simulink model "CyberDog_Motor_FOC"  (R2025b)
settings: Solver=FixedStepDiscrete  StartTime=0.0  StopTime=inf  FixedStep=0.0001  RelTol=1e-3
InitFcn:
  | p = fileparts(get_param(bdroot,'FileName')); addpath(fullfile(p,'scripts')); motor_params;
undefined symbols (not defined in the file): Cogging_Lut_Angle, Cogging_Lut_V, CoggingFF_En, Curr_MaxOut, Curr_MinOut, CurrD_Ki, CurrD_Kp, CurrD_MaxOut, CurrD_MinOut, CurrQ_Ki, CurrQ_Kp, DeadComp_En, DeadComp_Lut_I, DeadComp_Lut_V, InvTwoPiPolePairs, InvVbus, MotorCfg, PLL_Ki, PLL_Kp, Pos_Kd, Pos_Kp, Pos_MaxOut, Pos_MinOut, Speed_Ki, Speed_Kp, Speed_MaxOut, Speed_MinOut, VmaxCoeff
libraries: slpidlib x4, mcbeeMathTransformLib x3, mcbcontrolslib x2, mcbsensorlessestimatorlib x1
settings Model: Creator=Baseline  LastModifiedBy=Baseline
settings DataIOCC: SaveOutput=off
settings OptimizationCC: DefaultParameterBehavior=Inlined  DefaultUnderspecifiedDataType=single  EnhancedBackFolding=on  PassReuseOutputArgsAs=Individual arguments  ZeroExternalMemoryAtStartup=off  ZeroInternalMemoryAtStartup=off  OptimizeBlockOrder=speed  DifferentSizesBufferReuse=on  OptimizationCustomize=off  EfficientTunableParamExpr=on
settings DebuggingCC: ParameterPrecisionLossMsg=none  ParameterTunabilityLossMsg=error
settings SFSimCC: MATLABDynamicMemAlloc=off
settings RTWCC: SystemTargetFile=ert.tlc  GenCodeOnly=on  GenerateMakefile=off  TemplateMakefile=ert_default_tmf  Description=Embedded Coder
settings CodeAppCC: ForceParamTrailComments=on  IgnoreCustomStorageClasses=off  OperatorAnnotations=on  SimulinkDataObjDesc=on  SFDataObjDesc=on  InsertBlockDesc=on
settings ERTTargetCC: ERTCustomFileTemplate=example_file_process.tlc  TargetLangStandard=C99 (ISO)  GenerateSampleERTMain=on

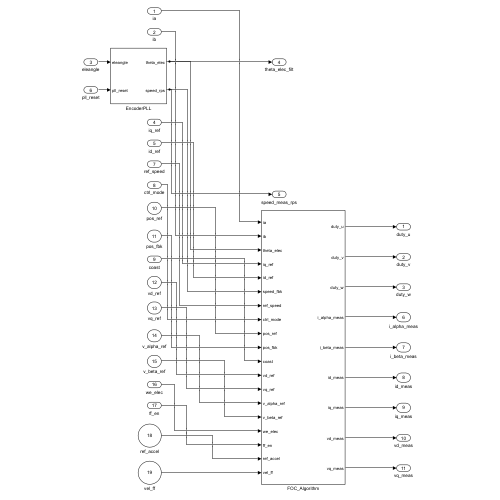
[thumbnail: Simulink's stored preview of the top-level diagram]
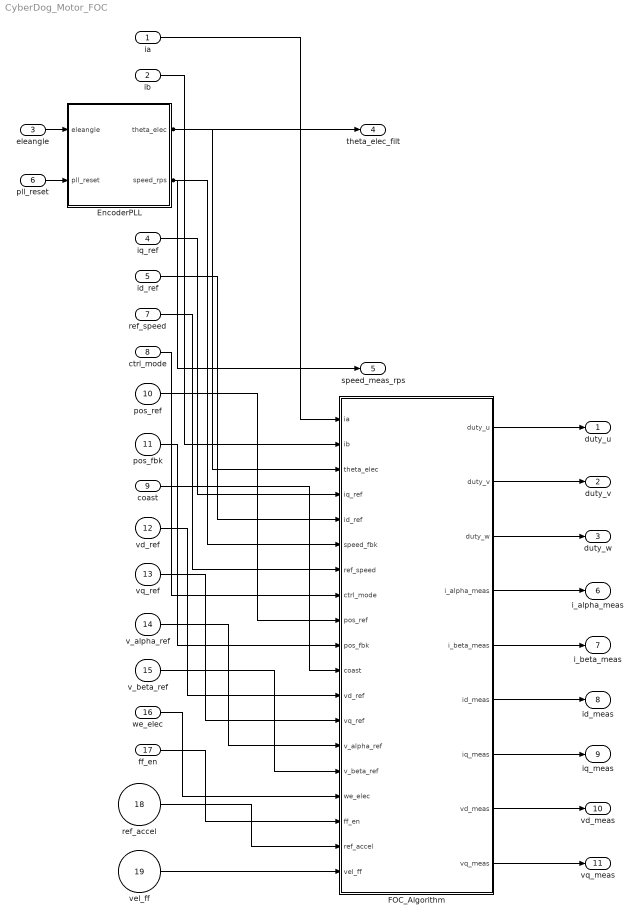
== system CyberDog_Motor_FOC ==
  ia : Inport  OutDataTypeStr=single  SampleTime=1e-4
  ib : Inport  Port=2  OutDataTypeStr=single  SampleTime=1e-4
  eleangle : Inport  Port=3  OutDataTypeStr=single  SampleTime=1e-4
  iq_ref : Inport  Port=4  OutDataTypeStr=single  SampleTime=1e-4
  id_ref : Inport  Port=5  OutDataTypeStr=single  SampleTime=1e-4
  pll_reset : Inport  Port=6  OutDataTypeStr=single  SampleTime=1e-4
  ref_speed : Inport  Port=7  OutDataTypeStr=single  SampleTime=1e-4
  ctrl_mode : Inport  Port=8  OutDataTypeStr=single  SampleTime=1e-4
  coast : Inport  Port=9  OutDataTypeStr=single
  pos_ref : Inport  Port=10  OutDataTypeStr=single
  pos_fbk : Inport  Port=11  OutDataTypeStr=single
  vd_ref : Inport  Port=12  OutDataTypeStr=single
  vq_ref : Inport  Port=13  OutDataTypeStr=single
  v_alpha_ref : Inport  Port=14  OutDataTypeStr=single
  v_beta_ref : Inport  Port=15  OutDataTypeStr=single
  we_elec : Inport  Port=16
  ff_en : Inport  Port=17
  ref_accel : Inport  Port=18
  vel_ff : Inport  Port=19
  EncoderPLL : Subsystem
  FOC_Algorithm : Subsystem
      settings: MinAlgLoopOccurrences=on
  duty_u : Outport  OutDataTypeStr=single
  duty_v : Outport  Port=2  OutDataTypeStr=single
  duty_w : Outport  Port=3  OutDataTypeStr=single
  theta_elec_filt : Outport  Port=4
  speed_meas_rps : Outport  Port=5
  i_alpha_meas : Outport  Port=6
  i_beta_meas : Outport  Port=7
  id_meas : Outport  Port=8
  iq_meas : Outport  Port=9
  vd_meas : Outport  Port=10
  vq_meas : Outport  Port=11
  wires:
  eleangle/1 -> EncoderPLL/1(eleangle)
  pll_reset/1 -> EncoderPLL/2(pll_reset)
  id_ref/1 -> FOC_Algorithm/5(id_ref)
  FOC_Algorithm/7(iq_meas) -> iq_meas/1
  EncoderPLL/1(theta_elec) -> theta_elec_filt/1, FOC_Algorithm/3(theta_elec)
  FOC_Algorithm/9(vq_meas) -> vq_meas/1
  FOC_Algorithm/5(i_beta_meas) -> i_beta_meas/1
  ia/1 -> FOC_Algorithm/1(ia)
  ib/1 -> FOC_Algorithm/2(ib)
  iq_ref/1 -> FOC_Algorithm/4(iq_ref)
  EncoderPLL/2(speed_rps) -> FOC_Algorithm/6(speed_fbk), speed_meas_rps/1
  coast/1 -> FOC_Algorithm/11(coast)
  ctrl_mode/1 -> FOC_Algorithm/8(ctrl_mode)
  ref_speed/1 -> FOC_Algorithm/7(ref_speed)
  pos_ref/1 -> FOC_Algorithm/9(pos_ref)
  FOC_Algorithm/8(vd_meas) -> vd_meas/1
  FOC_Algorithm/4(i_alpha_meas) -> i_alpha_meas/1
  pos_fbk/1 -> FOC_Algorithm/10(pos_fbk)
  vd_ref/1 -> FOC_Algorithm/12(vd_ref)
  FOC_Algorithm/1(duty_u) -> duty_u/1
  vq_ref/1 -> FOC_Algorithm/13(vq_ref)
  v_alpha_ref/1 -> FOC_Algorithm/14(v_alpha_ref)
  v_beta_ref/1 -> FOC_Algorithm/15(v_beta_ref)
  we_elec/1 -> FOC_Algorithm/16(we_elec)
  ff_en/1 -> FOC_Algorithm/17(ff_en)
  ref_accel/1 -> FOC_Algorithm/18(ref_accel)
  vel_ff/1 -> FOC_Algorithm/19(vel_ff)
  FOC_Algorithm/2(duty_v) -> duty_v/1
  FOC_Algorithm/3(duty_w) -> duty_w/1
  FOC_Algorithm/6(id_meas) -> id_meas/1

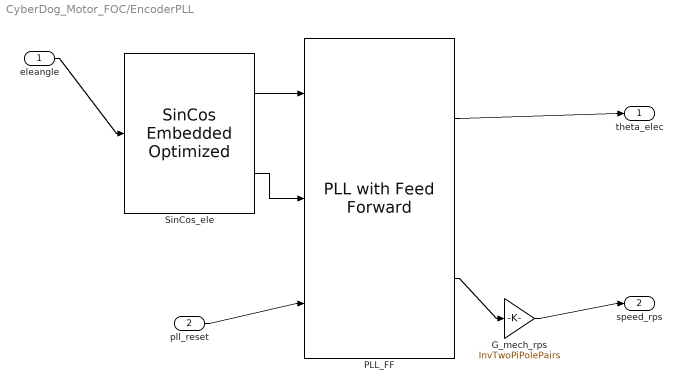
== system CyberDog_Motor_FOC/EncoderPLL ==
  eleangle : Inport
  pll_reset : Inport  Port=2
  G_mech_rps : Gain  Gain=InvTwoPiPolePairs
  PLL_FF : mcbsensorlessestimatorlib/PLL with Feed Forward  Normalization=off  ParameterBusInput=off  PosOut=Angular position  BlkSampleTime=1e-4  FreqRatio=1  MaximumApplicationFreq=7500  SpeedCutoffFreq=PLL_SpeedCutoffFreq  N_points=1024  Kp=PLL_Kp  Ki=PLL_Ki  PositionUnit=Radians  PositionDataType=single  FrequencyUnit=Radians/Sec  FrequencyDataType=single  TableDataType=single
      settings: LibrarySourceBlock=mcblib/Signal Management/PLL with Feed Forward
  SinCos_ele : mcbcontrolslib/SinCos Embedded Optimized  LabelModeActiveChoice=MCB_Sin  OptforProc=off  ApproximationMethod=None  UserApproxMethod=Lookup  ApproxStatus=None  InterpMethod=Linear point-slope  NumberOfDataPoints=16  NumberOfIterations=11  RemoveProtectionAgainstOutOfRangeInput=off  TableDataTypeStr=Inherit: Inherit via input  AngleInput=Radians  ThetaDataType=single  N_points=1024  DatatypeInput=Inherit from input  Datatype=single
  theta_elec : Outport
  speed_rps : Outport  Port=2
  wires:
  pll_reset/1 -> PLL_FF/3
  PLL_FF/1 -> theta_elec/1
  PLL_FF/2 -> G_mech_rps/1
  G_mech_rps/1 -> speed_rps/1
  eleangle/1 -> SinCos_ele/1
  SinCos_ele/1 -> PLL_FF/1
  SinCos_ele/2 -> PLL_FF/2

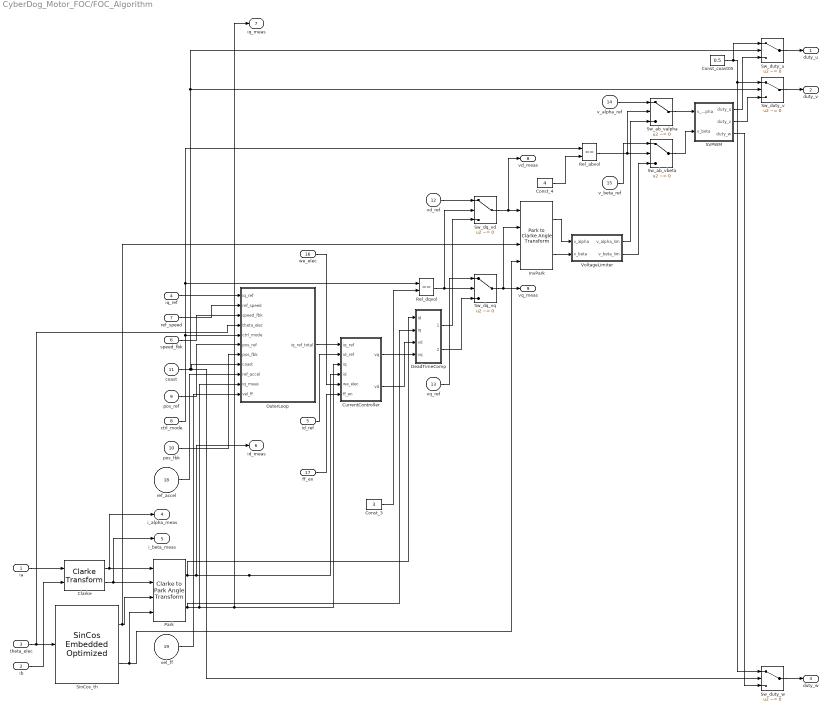
== system CyberDog_Motor_FOC/FOC_Algorithm ==
  ia : Inport
  ib : Inport  Port=2
  theta_elec : Inport  Port=3  OutDataTypeStr=single
  iq_ref : Inport  Port=4  OutDataTypeStr=single
  id_ref : Inport  Port=5  OutDataTypeStr=single
  speed_fbk : Inport  Port=6  OutDataTypeStr=single
  ref_speed : Inport  Port=7  OutDataTypeStr=single
  ctrl_mode : Inport  Port=8  OutDataTypeStr=single
  pos_ref : Inport  Port=9  OutDataTypeStr=single
  pos_fbk : Inport  Port=10  OutDataTypeStr=single
  coast : Inport  Port=11  OutDataTypeStr=single
  vd_ref : Inport  Port=12  OutDataTypeStr=single
  vq_ref : Inport  Port=13  OutDataTypeStr=single
  v_alpha_ref : Inport  Port=14  OutDataTypeStr=single
  v_beta_ref : Inport  Port=15  OutDataTypeStr=single
  we_elec : Inport  Port=16
  ff_en : Inport  Port=17
  ref_accel : Inport  Port=18
  vel_ff : Inport  Port=19
  Clarke : mcbeeMathTransformLib/Clarke Transform  VariantControl=Variant2  PowerInvariant=off  UseWithEmbedded=on  PhaseInput=Two inputs
      settings: LibrarySourceBlock=mcbfoclib/Field-Oriented Current Controller/Clarke Transform
  Const_3 : Constant  Value=3  OutDataTypeStr=single
  Const_4 : Constant  Value=4  OutDataTypeStr=single
  Const_coast05 : Constant  Value=0.5  OutDataTypeStr=single
  CurrentController : Subsystem
  DeadTimeComp : Subsystem
  InvPark : mcbeeMathTransformLib/Park to Clarke Angle Transform  AxisAlignment=D-axis  UseWithEmbedded=on  PhaseInput=Two inputs  ThetaInput=Sine and Cosine electrical position  AngleInput=Per-unit  N_points=1024
      settings: LibrarySourceBlock=mcbfoclib/Field-Oriented Current Controller/Inverse Park Transform
  OuterLoop : Subsystem
  Park : mcbeeMathTransformLib/Clarke to Park Angle Transform  AxisAlignment=D-axis  UseWithEmbedded=on  PhaseInput=Two inputs  ThetaInput=Sine and Cosine electrical position  AngleInput=Radians  N_points=1024
      settings: LibrarySourceBlock=mcbfoclib/Field-Oriented Current Controller/Park Transform
  Rel_abvol : RelationalOperator  Operator===  OutDataTypeStr=boolean  RndMeth=Simplest  InputSameDT=off
  Rel_dqvol : RelationalOperator  Operator===  OutDataTypeStr=boolean  RndMeth=Simplest  InputSameDT=off
  SVPWM : Subsystem
  SinCos_th : mcbcontrolslib/SinCos Embedded Optimized  LabelModeActiveChoice=MCB_Sin  OptforProc=off  ApproximationMethod=None  UserApproxMethod=Lookup  ApproxStatus=None  InterpMethod=Linear point-slope  NumberOfDataPoints=16  NumberOfIterations=11  RemoveProtectionAgainstOutOfRangeInput=off  TableDataTypeStr=Inherit: Inherit via input  AngleInput=Radians  ThetaDataType=single  N_points=1024  DatatypeInput=Inherit from input  Datatype=single
  Sw_ab_valpha : Switch  Criteria=u2 ~= 0  SaturateOnIntegerOverflow=off  InputSameDT=off
  Sw_ab_vbeta : Switch  Criteria=u2 ~= 0  SaturateOnIntegerOverflow=off  InputSameDT=off
  Sw_dq_vd : Switch  Criteria=u2 ~= 0  SaturateOnIntegerOverflow=off  InputSameDT=off
  Sw_dq_vq : Switch  Criteria=u2 ~= 0  SaturateOnIntegerOverflow=off  InputSameDT=off
  Sw_duty_u : Switch  Criteria=u2 ~= 0  SaturateOnIntegerOverflow=off  InputSameDT=off
  Sw_duty_v : Switch  Criteria=u2 ~= 0  SaturateOnIntegerOverflow=off  InputSameDT=off
  Sw_duty_w : Switch  Criteria=u2 ~= 0  SaturateOnIntegerOverflow=off  InputSameDT=off
  VoltageLimiter : Subsystem
  duty_u : Outport
  duty_v : Outport  Port=2
  duty_w : Outport  Port=3
  i_alpha_meas : Outport  Port=4
  i_beta_meas : Outport  Port=5
  id_meas : Outport  Port=6
  iq_meas : Outport  Port=7
  vd_meas : Outport  Port=8
  vq_meas : Outport  Port=9
  wires:
  ib/1 -> Clarke/2
  VoltageLimiter/2(v_beta_lim) -> Sw_ab_vbeta/3
  ctrl_mode/1 -> Rel_dqvol/1, Rel_abvol/1, OuterLoop/5(ctrl_mode)
  ia/1 -> Clarke/1
  Clarke/1 -> Park/1, i_alpha_meas/1
  vq_ref/1 -> Sw_dq_vq/1
  theta_elec/1 -> OuterLoop/4(theta_elec), SinCos_th/1
  iq_ref/1 -> OuterLoop/1(iq_ref)
  id_ref/1 -> CurrentController/2(id_ref)
  SinCos_th/1 -> InvPark/3, Park/3
  InvPark/1 -> VoltageLimiter/1(v_alpha)
  Clarke/2 -> Park/2, i_beta_meas/1
  Sw_dq_vq/1 -> vq_meas/1, InvPark/2
  SinCos_th/2 -> InvPark/4, Park/4
  ref_speed/1 -> OuterLoop/2(ref_speed)
  DeadTimeComp/1(vd_out) -> Sw_dq_vd/3
  speed_fbk/1 -> OuterLoop/3(speed_fbk)
  coast/1 -> Sw_duty_w/2, OuterLoop/8(coast), Sw_duty_u/2, Sw_duty_v/2
  pos_ref/1 -> OuterLoop/6(pos_ref)
  pos_fbk/1 -> OuterLoop/7(pos_fbk)
  ref_accel/1 -> OuterLoop/9(ref_accel)
  Park/1 -> CurrentController/4(id), id_meas/1, DeadTimeComp/1(id)
  Park/2 -> iq_meas/1, CurrentController/3(iq), OuterLoop/10(iq_meas), DeadTimeComp/2(iq)
  vel_ff/1 -> OuterLoop/11(vel_ff)
  SVPWM/1(duty_u) -> Sw_duty_u/3
  we_elec/1 -> CurrentController/5(we_elec)
  Sw_duty_u/1 -> duty_u/1
  Const_coast05/1 -> Sw_duty_v/1, Sw_duty_w/1, Sw_duty_u/1
  Const_3/1 -> Rel_dqvol/2
  OuterLoop/1(iq_ref_total) -> CurrentController/1(iq_ref)
  ff_en/1 -> CurrentController/6(ff_en)
  CurrentController/1(vq) -> DeadTimeComp/4(vq)
  v_beta_ref/1 -> Sw_ab_vbeta/1
  DeadTimeComp/2(vq_out) -> Sw_dq_vq/3
  CurrentController/2(vd) -> DeadTimeComp/3(vd)
  vd_ref/1 -> Sw_dq_vd/1
  Rel_dqvol/1 -> Sw_dq_vd/2, Sw_dq_vq/2
  Sw_dq_vd/1 -> vd_meas/1, InvPark/1
  Const_4/1 -> Rel_abvol/2
  InvPark/2 -> VoltageLimiter/2(v_beta)
  v_alpha_ref/1 -> Sw_ab_valpha/1
  Sw_duty_v/1 -> duty_v/1
  Rel_abvol/1 -> Sw_ab_vbeta/2, Sw_ab_valpha/2
  VoltageLimiter/1(v_alpha_lim) -> Sw_ab_valpha/3
  Sw_ab_valpha/1 -> SVPWM/1(v_alpha)
  Sw_ab_vbeta/1 -> SVPWM/2(v_beta)
  SVPWM/2(duty_v) -> Sw_duty_v/3
  SVPWM/3(duty_w) -> Sw_duty_w/3
  Sw_duty_w/1 -> duty_w/1

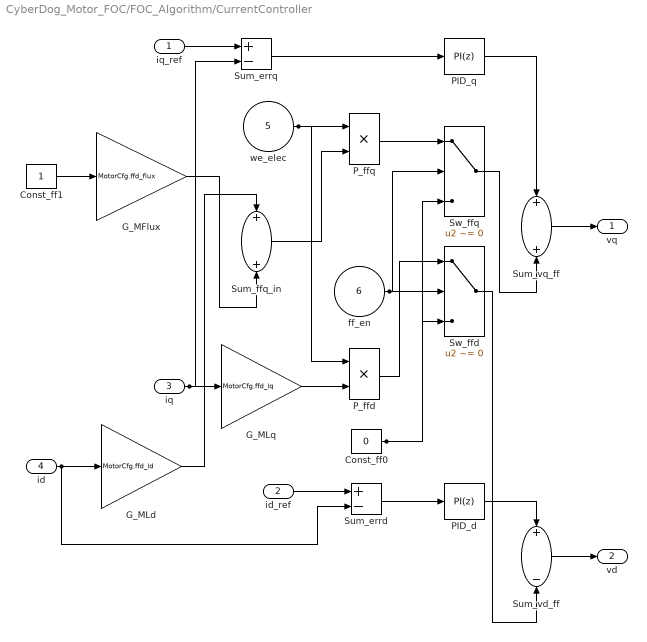
== system CyberDog_Motor_FOC/FOC_Algorithm/CurrentController ==
  iq_ref : Inport  OutDataTypeStr=single
  id_ref : Inport  Port=2  OutDataTypeStr=single
  iq : Inport  Port=3
  id : Inport  Port=4
  we_elec : Inport  Port=5
  ff_en : Inport  Port=6
  Const_ff0 : Constant  Value=0  OutDataTypeStr=single
  Const_ff1 : Constant  OutDataTypeStr=single
  G_MFlux : Gain  Gain=MotorCfg.ffd_flux  OutDataTypeStr=single
  G_MLd : Gain  Gain=MotorCfg.ffd_ld  OutDataTypeStr=single
  G_MLq : Gain  Gain=MotorCfg.ffd_lq  OutDataTypeStr=single
  PID_d : slpidlib/PID Controller  Controller=PI  Form=Parallel  TimeDomain=Discrete-time  UseExternalTs=off  SampleTime=1e-4  IntegratorMethod=Forward Euler  FilterMethod=Forward Euler  ControllerParametersSource=internal  P=CurrD_Kp  I=CurrD_Ki  UseKiTs=on  D=0  UseExternalDerivativeSource=off  N=100  UseFilter=on  TunerSelectOption=Transfer Function Based (PID Tuner App)  InitialConditionSource=internal  InitialConditionForIntegrator=0  InitialConditionForFilter=0  DifferentiatorICPrevScaledInput=0  ExternalReset=none  TrackingMode=off  Kt=1  LimitOutput=on  SatLimitsSource=internal  UpperSaturationLimit=CurrD_MaxOut  LowerSaturationLimit=CurrD_MinOut  LinearizeAsGain=on  AntiWindupMode=back-calculation  Kb=1  LimitIntegrator=on  UpperIntegratorSaturationLimit=CurrD_MaxOut  LowerIntegratorSaturationLimit=CurrD_MinOut  POutMin=[]  POutMax=[]  IOutMin=[]  IOutMax=[]  DOutMin=[]  DOutMax=[]  NOutMin=[]  NOutMax=[]  SumOutMin=[]  SumOutMax=[]  SaturationOutMin=[]  SaturationOutMax=[]  PParamDataTypeStr=single  PParamMin=[]  PParamMax=[]  IParamDataTypeStr=single  IParamMin=[]  IParamMax=[]  DParamMin=[]  DParamMax=[]  NParamMin=[]  NParamMax=[]  KbParamDataTypeStr=single  KbParamMin=[]  KbParamMax=[]  KtParamMin=[]  KtParamMax=[]  KbOutDataTypeStr=single  KbOutMin=[]  KbOutMax=[]  KtOutMin=[]  KtOutMax=[]  IntegratorOutMin=[]  IntegratorOutMax=[]  FilterOutMin=[]  FilterOutMax=[]  SumI1OutMin=[]  SumI1OutMax=[]  SumI2OutDataTypeStr=single  SumI2OutMin=[]  SumI2OutMax=[]  SumI3OutMin=[]  SumI3OutMax=[]  SumI4OutMin=[]  SumI4OutMax=[]  SumDOutMin=[]  SumDOutMax=[]  DifferentiatorOutMin=[]  DifferentiatorOutMax=[]  FilterDiffOutCoefMin=[]  FilterDiffOutCoefMax=[]  ReciprocalOutMin=[]  ReciprocalOutMax=[]  SumDenOutMin=[]  SumDenOutMax=[]  SumNumOutMin=[]  SumNumOutMax=[]  DivideOutMin=[]  DivideOutMax=[]  UdiffTsProdOutMin=[]  UdiffTsProdOutMax=[]  NTsProdOutMin=[]  NTsProdOutMax=[]  UintegralTsProdOutMin=[]  UintegralTsProdOutMax=[]  UngainTsProdOutMin=[]  UngainTsProdOutMax=[]  ClampingZeroOutDataTypeStr=Inherit: Inherit via back propagation  ClampingZeroOutMin=[]  ClampingZeroOutMax=[]  FilterDenConstantOutDataTypeStr=Inherit: Inherit via back propagation  FilterDenConstantOutMin=[]  FilterDenConstantOutMax=[]  PCopyOutDataTypeStr=Inherit: Inherit via back propagation  PCopyOutMin=[]  PCopyOutMax=[]  NCopyOutDataTypeStr=Inherit: Inherit via back propagation  NCopyOutMin=[]  NCopyOutMax=[]  IntegratorContinuousStateAttributes=''  IntegratorStateMustResolveToSignalObject=off  IntegratorRTWStateStorageClass=Auto  FilterContinuousStateAttributes=''  FilterStateMustResolveToSignalObject=off  FilterRTWStateStorageClass=Auto  ParallelPVariant=InternalParameters  IdealPVariant=Disabled  IVariant=InternalParameters  DVariant=Disabled  IntegratorVariant=Discrete  SatVariant=Enabled  AWVariant=BackCalculation  PCopyVariant=Disabled  TRVariant=Disabled  FdbkBlocksVariant=Forward  IdealPFdbkVariant=Disabled  SatFdbkVariant=Disabled  DerivativeFilterVariant=Disabled  NVariant=Disabled  NCopyVariant=Disabled_SignalSpec  FilterICVariant=Disabled  IntegratorICVariant=InternalICs  ExternalResetVariant=Disabled  TRSumVariant=Passthrough  SumFdbkVariant=Disabled  SumVariant=Sum_PI  TsampFilterVariant=InternalTs  TsampNgainVariant=Passthrough  TsampIntegralVariant=Disabled_SignalSpec  ExternalSaturationOutDataTypeStr=Inherit: Same as second input  DerivativeSourceVariant=Disabled  PreIntVariant=InternalPreInt
  PID_q : slpidlib/PID Controller  Controller=PI  Form=Parallel  TimeDomain=Discrete-time  UseExternalTs=off  SampleTime=1e-4  IntegratorMethod=Forward Euler  FilterMethod=Forward Euler  ControllerParametersSource=internal  P=CurrQ_Kp  I=CurrQ_Ki  UseKiTs=on  D=0  UseExternalDerivativeSource=off  N=100  UseFilter=on  TunerSelectOption=Transfer Function Based (PID Tuner App)  InitialConditionSource=internal  InitialConditionForIntegrator=0  InitialConditionForFilter=0  DifferentiatorICPrevScaledInput=0  ExternalReset=none  TrackingMode=off  Kt=1  LimitOutput=on  SatLimitsSource=internal  UpperSaturationLimit=Curr_MaxOut  LowerSaturationLimit=Curr_MinOut  LinearizeAsGain=on  AntiWindupMode=back-calculation  Kb=1  LimitIntegrator=on  UpperIntegratorSaturationLimit=Curr_MaxOut  LowerIntegratorSaturationLimit=Curr_MinOut  POutMin=[]  POutMax=[]  IOutMin=[]  IOutMax=[]  DOutMin=[]  DOutMax=[]  NOutMin=[]  NOutMax=[]  SumOutMin=[]  SumOutMax=[]  SaturationOutMin=[]  SaturationOutMax=[]  PParamDataTypeStr=single  PParamMin=[]  PParamMax=[]  IParamDataTypeStr=single  IParamMin=[]  IParamMax=[]  DParamMin=[]  DParamMax=[]  NParamMin=[]  NParamMax=[]  KbParamDataTypeStr=single  KbParamMin=[]  KbParamMax=[]  KtParamMin=[]  KtParamMax=[]  KbOutDataTypeStr=single  KbOutMin=[]  KbOutMax=[]  KtOutMin=[]  KtOutMax=[]  IntegratorOutMin=[]  IntegratorOutMax=[]  FilterOutMin=[]  FilterOutMax=[]  SumI1OutMin=[]  SumI1OutMax=[]  SumI2OutDataTypeStr=single  SumI2OutMin=[]  SumI2OutMax=[]  SumI3OutMin=[]  SumI3OutMax=[]  SumI4OutMin=[]  SumI4OutMax=[]  SumDOutMin=[]  SumDOutMax=[]  DifferentiatorOutMin=[]  DifferentiatorOutMax=[]  FilterDiffOutCoefMin=[]  FilterDiffOutCoefMax=[]  ReciprocalOutMin=[]  ReciprocalOutMax=[]  SumDenOutMin=[]  SumDenOutMax=[]  SumNumOutMin=[]  SumNumOutMax=[]  DivideOutMin=[]  DivideOutMax=[]  UdiffTsProdOutMin=[]  UdiffTsProdOutMax=[]  NTsProdOutMin=[]  NTsProdOutMax=[]  UintegralTsProdOutMin=[]  UintegralTsProdOutMax=[]  UngainTsProdOutMin=[]  UngainTsProdOutMax=[]  ClampingZeroOutDataTypeStr=Inherit: Inherit via back propagation  ClampingZeroOutMin=[]  ClampingZeroOutMax=[]  FilterDenConstantOutDataTypeStr=Inherit: Inherit via back propagation  FilterDenConstantOutMin=[]  FilterDenConstantOutMax=[]  PCopyOutDataTypeStr=Inherit: Inherit via back propagation  PCopyOutMin=[]  PCopyOutMax=[]  NCopyOutDataTypeStr=Inherit: Inherit via back propagation  NCopyOutMin=[]  NCopyOutMax=[]  IntegratorContinuousStateAttributes=''  IntegratorStateMustResolveToSignalObject=off  IntegratorRTWStateStorageClass=Auto  FilterContinuousStateAttributes=''  FilterStateMustResolveToSignalObject=off  FilterRTWStateStorageClass=Auto  ParallelPVariant=InternalParameters  IdealPVariant=Disabled  IVariant=InternalParameters  DVariant=Disabled  IntegratorVariant=Discrete  SatVariant=Enabled  AWVariant=BackCalculation  PCopyVariant=Disabled  TRVariant=Disabled  FdbkBlocksVariant=Forward  IdealPFdbkVariant=Disabled  SatFdbkVariant=Disabled  DerivativeFilterVariant=Disabled  NVariant=Disabled  NCopyVariant=Disabled_SignalSpec  FilterICVariant=Disabled  IntegratorICVariant=InternalICs  ExternalResetVariant=Disabled  TRSumVariant=Passthrough  SumFdbkVariant=Disabled  SumVariant=Sum_PI  TsampFilterVariant=InternalTs  TsampNgainVariant=Passthrough  TsampIntegralVariant=Disabled_SignalSpec  ExternalSaturationOutDataTypeStr=Inherit: Same as second input  DerivativeSourceVariant=Disabled  PreIntVariant=InternalPreInt
  P_ffd : Product  OutDataTypeStr=single
  P_ffq : Product  OutDataTypeStr=single
  Sum_errd : Sum  Inputs=+-
  Sum_errq : Sum  Inputs=+-
  Sum_ffq_in : Sum  OutDataTypeStr=single
  Sum_vd_ff : Sum  Inputs=+-  OutDataTypeStr=single
  Sum_vq_ff : Sum  OutDataTypeStr=single
  Sw_ffd : Switch  Criteria=u2 ~= 0  OutDataTypeStr=single
  Sw_ffq : Switch  Criteria=u2 ~= 0  OutDataTypeStr=single
  vq : Outport
  vd : Outport  Port=2
  wires:
  Sum_errq/1 -> PID_q/1
  G_MLd/1 -> Sum_ffq_in/1
  Const_ff1/1 -> G_MFlux/1
  G_MFlux/1 -> Sum_ffq_in/2
  id/1 -> Sum_errd/2, G_MLd/1
  iq_ref/1 -> Sum_errq/1
  iq/1 -> G_MLq/1, Sum_errq/2
  we_elec/1 -> P_ffd/1, P_ffq/1
  Const_ff0/1 -> Sw_ffd/3, Sw_ffq/3
  Sum_ffq_in/1 -> P_ffq/2
  G_MLq/1 -> P_ffd/2
  id_ref/1 -> Sum_errd/1
  P_ffd/1 -> Sw_ffd/1
  P_ffq/1 -> Sw_ffq/1
  ff_en/1 -> Sw_ffd/2, Sw_ffq/2
  Sum_errd/1 -> PID_d/1
  PID_q/1 -> Sum_vq_ff/1
  Sw_ffq/1 -> Sum_vq_ff/2
  Sw_ffd/1 -> Sum_vd_ff/2
  PID_d/1 -> Sum_vd_ff/1
  Sum_vd_ff/1 -> vd/1
  Sum_vq_ff/1 -> vq/1

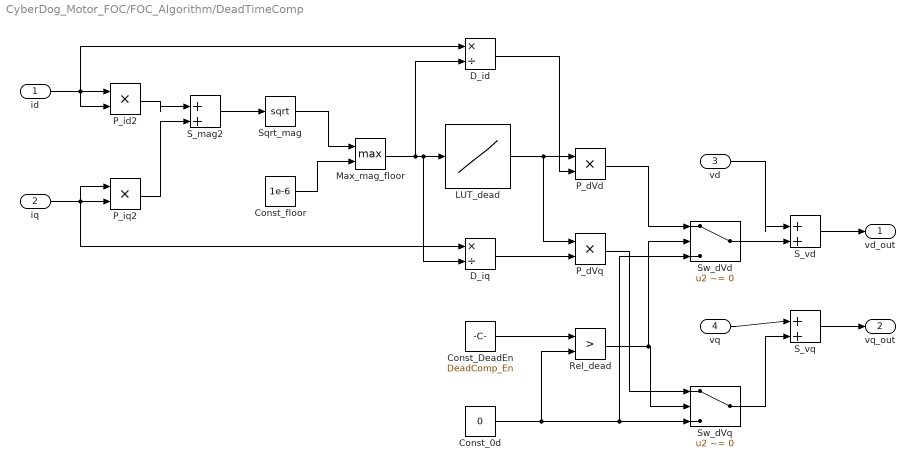
== system CyberDog_Motor_FOC/FOC_Algorithm/DeadTimeComp ==
  id : Inport
  iq : Inport  Port=2
  vd : Inport  Port=3
  vq : Inport  Port=4
  Const_0d : Constant  Value=0  OutDataTypeStr=single
  Const_DeadEn : Constant  Value=DeadComp_En  OutDataTypeStr=single
  Const_floor : Constant  Value=1e-6  OutDataTypeStr=single
  D_id : Product  Inputs=*/  OutDataTypeStr=single
  D_iq : Product  Inputs=*/  OutDataTypeStr=single
  LUT_dead : Lookup_n-D  NumberOfTableDimensions=1  BreakpointsForDimension1=DeadComp_Lut_I  Table=DeadComp_Lut_V  InternalRulePriority=Speed  OutDataTypeStr=single  RndMeth=Simplest
  Max_mag_floor : MinMax  Function=max  Inputs=2  OutDataTypeStr=single
  P_dVd : Product  Inputs=**  OutDataTypeStr=single
  P_dVq : Product  Inputs=**  OutDataTypeStr=single
  P_id2 : Product  Inputs=**  OutDataTypeStr=single
  P_iq2 : Product  Inputs=**  OutDataTypeStr=single
  Rel_dead : RelationalOperator  Operator=>  OutDataTypeStr=boolean  RndMeth=Simplest  InputSameDT=off
  S_mag2 : Sum  Inputs=|++  OutDataTypeStr=single
  S_vd : Sum  Inputs=|++
  S_vq : Sum  Inputs=|++
  Sqrt_mag : Sqrt  OutDataTypeStr=single
  Sw_dVd : Switch  Criteria=u2 ~= 0  OutDataTypeStr=single  SaturateOnIntegerOverflow=off  InputSameDT=off
  Sw_dVq : Switch  Criteria=u2 ~= 0  OutDataTypeStr=single  SaturateOnIntegerOverflow=off  InputSameDT=off
  vd_out : Outport
  vq_out : Outport  Port=2
  wires:
  S_vq/1 -> vq_out/1
  S_vd/1 -> vd_out/1
  Sw_dVq/1 -> S_vq/2
  vq/1 -> S_vq/1
  Sw_dVd/1 -> S_vd/2
  vd/1 -> S_vd/1
  Const_DeadEn/1 -> Rel_dead/1
  P_dVq/1 -> Sw_dVq/1
  Const_0d/1 -> Sw_dVd/3, Sw_dVq/3, Rel_dead/2
  Rel_dead/1 -> Sw_dVd/2, Sw_dVq/2
  P_dVd/1 -> Sw_dVd/1
  D_iq/1 -> P_dVq/2
  D_id/1 -> P_dVd/2
  LUT_dead/1 -> P_dVd/1, P_dVq/1
  Max_mag_floor/1 -> LUT_dead/1, D_iq/2, D_id/2
  Const_floor/1 -> Max_mag_floor/2
  Sqrt_mag/1 -> Max_mag_floor/1
  S_mag2/1 -> Sqrt_mag/1
  P_iq2/1 -> S_mag2/2
  P_id2/1 -> S_mag2/1
  iq/1 -> D_iq/1, P_iq2/1, P_iq2/2
  id/1 -> P_id2/1, P_id2/2, D_id/1

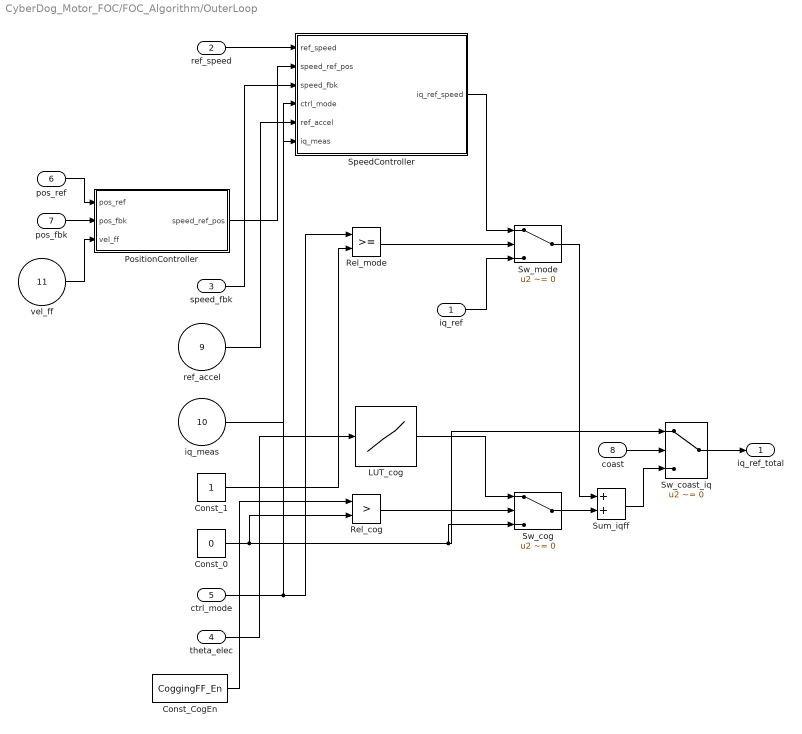
== system CyberDog_Motor_FOC/FOC_Algorithm/OuterLoop ==
  iq_ref : Inport  OutDataTypeStr=single
  ref_speed : Inport  Port=2  OutDataTypeStr=single
  speed_fbk : Inport  Port=3  OutDataTypeStr=single
  theta_elec : Inport  Port=4  OutDataTypeStr=single
  ctrl_mode : Inport  Port=5  OutDataTypeStr=single
  pos_ref : Inport  Port=6  OutDataTypeStr=single
  pos_fbk : Inport  Port=7  OutDataTypeStr=single
  coast : Inport  Port=8  OutDataTypeStr=single
  ref_accel : Inport  Port=9
  iq_meas : Inport  Port=10
  vel_ff : Inport  Port=11
  Const_0 : Constant  Value=0  OutDataTypeStr=single
  Const_1 : Constant  OutDataTypeStr=single
  Const_CogEn : Constant  Value=CoggingFF_En  OutDataTypeStr=single
  LUT_cog : Lookup_n-D  NumberOfTableDimensions=1  BreakpointsForDimension1=Cogging_Lut_Angle  Table=Cogging_Lut_V  InternalRulePriority=Speed  OutDataTypeStr=single  RndMeth=Simplest
  PositionController : Subsystem
  Rel_cog : RelationalOperator  Operator=>  OutDataTypeStr=boolean  RndMeth=Simplest  InputSameDT=off
  Rel_mode : RelationalOperator  OutDataTypeStr=boolean  RndMeth=Simplest  InputSameDT=off
  SpeedController : Subsystem
  Sum_iqff : Sum  OutDataTypeStr=single
  Sw_coast_iq : Switch  Criteria=u2 ~= 0  SaturateOnIntegerOverflow=off  InputSameDT=off
  Sw_cog : Switch  Criteria=u2 ~= 0  OutDataTypeStr=single  SaturateOnIntegerOverflow=off  InputSameDT=off
  Sw_mode : Switch  Criteria=u2 ~= 0  OutDataTypeStr=single  SaturateOnIntegerOverflow=off  InputSameDT=off
  iq_ref_total : Outport
  wires:
  Sw_cog/1 -> Sum_iqff/2
  pos_fbk/1 -> PositionController/2(pos_fbk)
  speed_fbk/1 -> SpeedController/3(speed_fbk)
  pos_ref/1 -> PositionController/1(pos_ref)
  ref_speed/1 -> SpeedController/1(ref_speed)
  vel_ff/1 -> PositionController/3(vel_ff)
  LUT_cog/1 -> Sw_cog/1
  iq_meas/1 -> SpeedController/6(iq_meas)
  PositionController/1(speed_ref_pos) -> SpeedController/2(speed_ref_pos)
  ref_accel/1 -> SpeedController/5(ref_accel)
  Const_1/1 -> Rel_mode/2
  Sw_mode/1 -> Sum_iqff/1
  Const_0/1 -> Sw_cog/3, Sw_coast_iq/1, Rel_cog/2
  iq_ref/1 -> Sw_mode/3
  ctrl_mode/1 -> Rel_mode/1, SpeedController/4(ctrl_mode)
  theta_elec/1 -> LUT_cog/1
  Const_CogEn/1 -> Rel_cog/1
  SpeedController/1(iq_ref_speed) -> Sw_mode/1
  Rel_mode/1 -> Sw_mode/2
  Rel_cog/1 -> Sw_cog/2
  coast/1 -> Sw_coast_iq/2
  Sum_iqff/1 -> Sw_coast_iq/3
  Sw_coast_iq/1 -> iq_ref_total/1

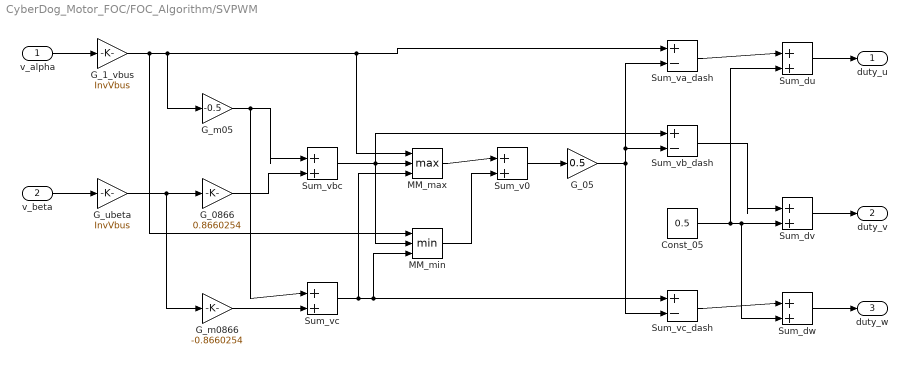
== system CyberDog_Motor_FOC/FOC_Algorithm/SVPWM ==
  v_alpha : Inport  OutDataTypeStr=single
  v_beta : Inport  Port=2  OutDataTypeStr=single
  Const_05 : Constant  Value=0.5  OutDataTypeStr=single
  G_05 : Gain  Gain=0.5  ParamDataTypeStr=single  OutDataTypeStr=single
  G_0866 : Gain  Gain=0.8660254  ParamDataTypeStr=single  OutDataTypeStr=single
  G_1_vbus : Gain  Gain=InvVbus  ParamDataTypeStr=single  OutDataTypeStr=single
  G_m05 : Gain  Gain=-0.5  ParamDataTypeStr=single  OutDataTypeStr=single
  G_m0866 : Gain  Gain=-0.8660254  ParamDataTypeStr=single  OutDataTypeStr=single
  G_ubeta : Gain  Gain=InvVbus  ParamDataTypeStr=single  OutDataTypeStr=single
  MM_max : MinMax  Function=max  Inputs=3  OutDataTypeStr=single
  MM_min : MinMax  Inputs=3  OutDataTypeStr=single
  Sum_du : Sum  Inputs=|++  OutDataTypeStr=single
  Sum_dv : Sum  Inputs=|++  OutDataTypeStr=single
  Sum_dw : Sum  Inputs=|++  OutDataTypeStr=single
  Sum_v0 : Sum  Inputs=|++  OutDataTypeStr=single
  Sum_va_dash : Sum  Inputs=+-  OutDataTypeStr=single
  Sum_vb_dash : Sum  Inputs=+-  OutDataTypeStr=single
  Sum_vbc : Sum  Inputs=|++  OutDataTypeStr=single
  Sum_vc : Sum  Inputs=|++  OutDataTypeStr=single
  Sum_vc_dash : Sum  Inputs=+-  OutDataTypeStr=single
  duty_u : Outport
  duty_v : Outport  Port=2
  duty_w : Outport  Port=3
  wires:
  Sum_dw/1 -> duty_w/1
  Sum_dv/1 -> duty_v/1
  Sum_du/1 -> duty_u/1
  Sum_vc_dash/1 -> Sum_dw/1
  Sum_vb_dash/1 -> Sum_dv/1
  Const_05/1 -> Sum_dv/2, Sum_dw/2, Sum_du/2
  Sum_va_dash/1 -> Sum_du/1
  G_05/1 -> Sum_va_dash/2, Sum_vb_dash/2, Sum_vc_dash/2
  Sum_v0/1 -> G_05/1
  MM_min/1 -> Sum_v0/2
  MM_max/1 -> Sum_v0/1
  Sum_vc/1 -> Sum_vc_dash/1, MM_min/3, MM_max/3
  Sum_vbc/1 -> MM_max/2, MM_min/2, Sum_vb_dash/1
  G_m0866/1 -> Sum_vc/2
  G_0866/1 -> Sum_vbc/2
  G_m05/1 -> Sum_vbc/1, Sum_vc/1
  G_ubeta/1 -> G_0866/1, G_m0866/1
  G_1_vbus/1 -> Sum_va_dash/1, MM_max/1, G_m05/1, MM_min/1
  v_beta/1 -> G_ubeta/1
  v_alpha/1 -> G_1_vbus/1

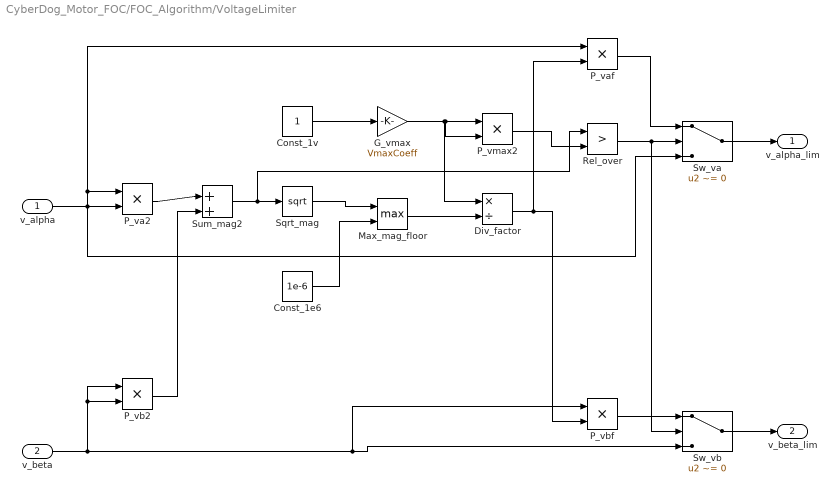
== system CyberDog_Motor_FOC/FOC_Algorithm/VoltageLimiter ==
  v_alpha : Inport
  v_beta : Inport  Port=2
  Const_1e6 : Constant  Value=1e-6  OutDataTypeStr=single
  Const_1v : Constant  OutDataTypeStr=single
  Div_factor : Product  Inputs=*/  OutDataTypeStr=single
  G_vmax : Gain  Gain=VmaxCoeff  ParamDataTypeStr=single  OutDataTypeStr=single
  Max_mag_floor : MinMax  Function=max  Inputs=2  OutDataTypeStr=single
  P_va2 : Product  Inputs=**  OutDataTypeStr=single
  P_vaf : Product  Inputs=**  OutDataTypeStr=single
  P_vb2 : Product  Inputs=**  OutDataTypeStr=single
  P_vbf : Product  Inputs=**  OutDataTypeStr=single
  P_vmax2 : Product  Inputs=**  OutDataTypeStr=single
  Rel_over : RelationalOperator  Operator=>  OutDataTypeStr=boolean  RndMeth=Simplest  InputSameDT=off
  Sqrt_mag : Sqrt  OutDataTypeStr=single
  Sum_mag2 : Sum  Inputs=|++  OutDataTypeStr=single
  Sw_va : Switch  Criteria=u2 ~= 0  OutDataTypeStr=single  SaturateOnIntegerOverflow=off  InputSameDT=off
  Sw_vb : Switch  Criteria=u2 ~= 0  OutDataTypeStr=single  SaturateOnIntegerOverflow=off  InputSameDT=off
  v_alpha_lim : Outport
  v_beta_lim : Outport  Port=2
  wires:
  Sw_vb/1 -> v_beta_lim/1
  Sw_va/1 -> v_alpha_lim/1
  P_vbf/1 -> Sw_vb/1
  Rel_over/1 -> Sw_va/2, Sw_vb/2
  P_vaf/1 -> Sw_va/1
  Div_factor/1 -> P_vaf/2, P_vbf/2
  Max_mag_floor/1 -> Div_factor/2
  Const_1e6/1 -> Max_mag_floor/2
  Sqrt_mag/1 -> Max_mag_floor/1
  P_vmax2/1 -> Rel_over/2
  Sum_mag2/1 -> Rel_over/1, Sqrt_mag/1
  P_vb2/1 -> Sum_mag2/2
  P_va2/1 -> Sum_mag2/1
  v_beta/1 -> P_vbf/1, Sw_vb/3, P_vb2/1, P_vb2/2
  v_alpha/1 -> P_va2/1, P_vaf/1, P_va2/2, Sw_va/3
  G_vmax/1 -> P_vmax2/2, P_vmax2/1, Div_factor/1
  Const_1v/1 -> G_vmax/1

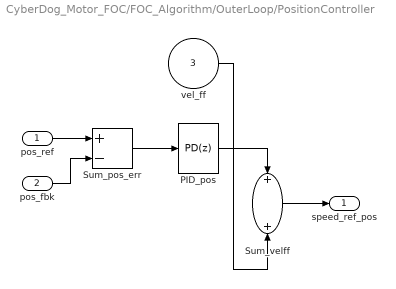
== system CyberDog_Motor_FOC/FOC_Algorithm/OuterLoop/PositionController ==
  pos_ref : Inport
  pos_fbk : Inport  Port=2
  vel_ff : Inport  Port=3
  PID_pos : slpidlib/PID Controller  Controller=PD  Form=Parallel  TimeDomain=Discrete-time  UseExternalTs=off  SampleTime=1e-3  IntegratorMethod=Forward Euler  FilterMethod=Forward Euler  ControllerParametersSource=internal  P=Pos_Kp  I=1  UseKiTs=off  D=Pos_Kd  UseExternalDerivativeSource=off  N=100  UseFilter=on  TunerSelectOption=Transfer Function Based (PID Tuner App)  InitialConditionSource=internal  InitialConditionForIntegrator=0  InitialConditionForFilter=0  DifferentiatorICPrevScaledInput=0  ExternalReset=none  TrackingMode=off  Kt=1  LimitOutput=on  SatLimitsSource=internal  UpperSaturationLimit=Pos_MaxOut  LowerSaturationLimit=Pos_MinOut  LinearizeAsGain=on  AntiWindupMode=none  Kb=1  LimitIntegrator=off  UpperIntegratorSaturationLimit=inf  LowerIntegratorSaturationLimit=-inf  POutMin=[]  POutMax=[]  IOutMin=[]  IOutMax=[]  DOutMin=[]  DOutMax=[]  NOutMin=[]  NOutMax=[]  SumOutMin=[]  SumOutMax=[]  SaturationOutMin=[]  SaturationOutMax=[]  PParamMin=[]  PParamMax=[]  IParamMin=[]  IParamMax=[]  DParamMin=[]  DParamMax=[]  NParamMin=[]  NParamMax=[]  KbParamMin=[]  KbParamMax=[]  KtParamMin=[]  KtParamMax=[]  KbOutMin=[]  KbOutMax=[]  KtOutMin=[]  KtOutMax=[]  IntegratorOutMin=[]  IntegratorOutMax=[]  FilterOutMin=[]  FilterOutMax=[]  SumI1OutMin=[]  SumI1OutMax=[]  SumI2OutMin=[]  SumI2OutMax=[]  SumI3OutMin=[]  SumI3OutMax=[]  SumI4OutMin=[]  SumI4OutMax=[]  SumDOutMin=[]  SumDOutMax=[]  DifferentiatorOutMin=[]  DifferentiatorOutMax=[]  FilterDiffOutCoefMin=[]  FilterDiffOutCoefMax=[]  ReciprocalOutMin=[]  ReciprocalOutMax=[]  SumDenOutMin=[]  SumDenOutMax=[]  SumNumOutMin=[]  SumNumOutMax=[]  DivideOutMin=[]  DivideOutMax=[]  UdiffTsProdOutMin=[]  UdiffTsProdOutMax=[]  NTsProdOutMin=[]  NTsProdOutMax=[]  UintegralTsProdOutMin=[]  UintegralTsProdOutMax=[]  UngainTsProdOutMin=[]  UngainTsProdOutMax=[]  ClampingZeroOutDataTypeStr=Inherit: Inherit via back propagation  ClampingZeroOutMin=[]  ClampingZeroOutMax=[]  FilterDenConstantOutDataTypeStr=Inherit: Inherit via back propagation  FilterDenConstantOutMin=[]  FilterDenConstantOutMax=[]  PCopyOutDataTypeStr=Inherit: Inherit via back propagation  PCopyOutMin=[]  PCopyOutMax=[]  NCopyOutDataTypeStr=Inherit: Inherit via back propagation  NCopyOutMin=[]  NCopyOutMax=[]  IntegratorContinuousStateAttributes=''  IntegratorStateMustResolveToSignalObject=off  IntegratorRTWStateStorageClass=Auto  FilterContinuousStateAttributes=''  FilterStateMustResolveToSignalObject=off  FilterRTWStateStorageClass=Auto  ParallelPVariant=InternalParameters  IdealPVariant=Disabled  IVariant=Disabled  DVariant=InternalParameters  IntegratorVariant=Disabled  SatVariant=Enabled  AWVariant=Disabled  PCopyVariant=Disabled  TRVariant=Disabled  FdbkBlocksVariant=Forward  IdealPFdbkVariant=Disabled  SatFdbkVariant=Disabled  DerivativeFilterVariant=ForwardEulerFilter  NVariant=InternalParameters  NCopyVariant=Disabled  FilterICVariant=InternalICsFilter  IntegratorICVariant=Disabled  ExternalResetVariant=Disabled  TRSumVariant=Passthrough  SumFdbkVariant=Disabled  SumVariant=Sum_PD  TsampFilterVariant=InternalTs  TsampNgainVariant=Passthrough  TsampIntegralVariant=Disabled_SignalSpec  ExternalSaturationOutDataTypeStr=Inherit: Same as second input  DerivativeSourceVariant=ErrorSignal  PreIntVariant=InternalPreInt
  Sum_pos_err : Sum  Inputs=+-
  Sum_velff : Sum  OutDataTypeStr=single
  speed_ref_pos : Outport
  wires:
  Sum_velff/1 -> speed_ref_pos/1
  vel_ff/1 -> Sum_velff/2
  pos_fbk/1 -> Sum_pos_err/2
  pos_ref/1 -> Sum_pos_err/1
  PID_pos/1 -> Sum_velff/1
  Sum_pos_err/1 -> PID_pos/1

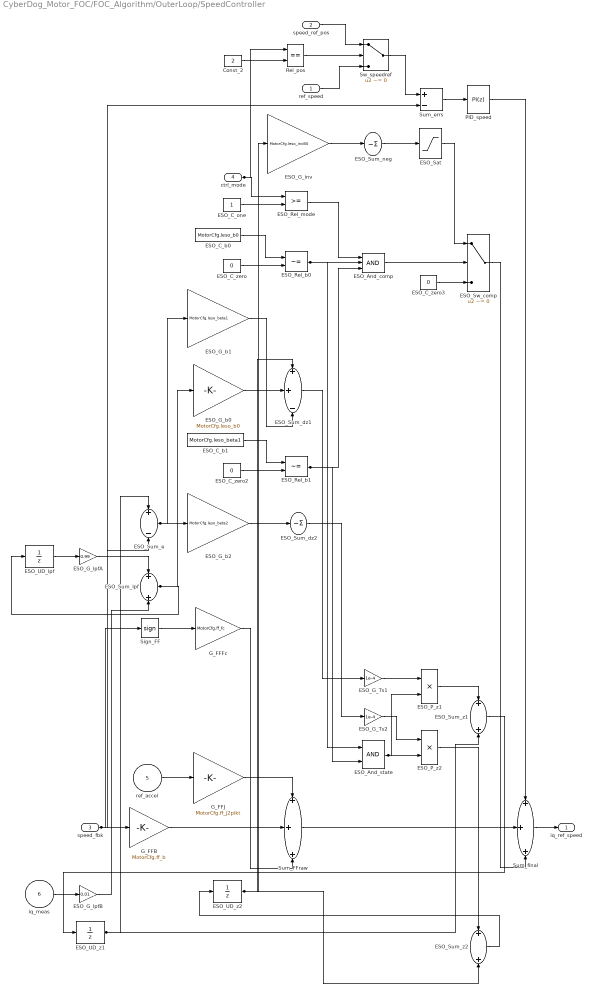
== system CyberDog_Motor_FOC/FOC_Algorithm/OuterLoop/SpeedController ==
  ref_speed : Inport
  speed_ref_pos : Inport  Port=2
  speed_fbk : Inport  Port=3
  ctrl_mode : Inport  Port=4
  ref_accel : Inport  Port=5
  iq_meas : Inport  Port=6
  Const_2 : Constant  Value=2  OutDataTypeStr=single
  ESO_And_comp : Logic  Inputs=3  AllPortsSameDT=off  OutDataTypeStr=boolean
  ESO_And_state : Logic  AllPortsSameDT=off  OutDataTypeStr=boolean
  ESO_C_b0 : Constant  Value=MotorCfg.leso_b0  OutDataTypeStr=single
  ESO_C_b1 : Constant  Value=MotorCfg.leso_beta1  OutDataTypeStr=single
  ESO_C_one : Constant  OutDataTypeStr=single
  ESO_C_zero : Constant  Value=0  OutDataTypeStr=single
  ESO_C_zero2 : Constant  Value=0  OutDataTypeStr=single
  ESO_C_zero3 : Constant  Value=0  OutDataTypeStr=single
  ESO_G_Ts1 : Gain  Gain=1e-4  OutDataTypeStr=single
  ESO_G_Ts2 : Gain  Gain=1e-4  OutDataTypeStr=single
  ESO_G_b0 : Gain  Gain=MotorCfg.leso_b0  OutDataTypeStr=single
  ESO_G_b1 : Gain  Gain=MotorCfg.leso_beta1  OutDataTypeStr=single
  ESO_G_b2 : Gain  Gain=MotorCfg.leso_beta2  OutDataTypeStr=single
  ESO_G_inv : Gain  Gain=MotorCfg.leso_invB0  OutDataTypeStr=single
  ESO_G_lpfA : Gain  Gain=0.99  OutDataTypeStr=single
  ESO_G_lpfB : Gain  Gain=0.01  OutDataTypeStr=single
  ESO_P_z1 : Product  OutDataTypeStr=single
  ESO_P_z2 : Product  OutDataTypeStr=single
  ESO_Rel_b0 : RelationalOperator  Operator=~=
  ESO_Rel_b1 : RelationalOperator  Operator=~=
  ESO_Rel_mode : RelationalOperator
  ESO_Sat : Saturate  UpperLimit=3  LowerLimit=-3  OutDataTypeStr=single
  ESO_Sum_dz1 : Sum  Inputs=++-  OutDataTypeStr=single
  ESO_Sum_dz2 : Sum  Inputs=-  OutDataTypeStr=single
  ESO_Sum_e : Sum  Inputs=+-  OutDataTypeStr=single
  ESO_Sum_lpf : Sum  OutDataTypeStr=single
  ESO_Sum_neg : Sum  Inputs=-  OutDataTypeStr=single
  ESO_Sum_z1 : Sum  OutDataTypeStr=single
  ESO_Sum_z2 : Sum  OutDataTypeStr=single
  ESO_Sw_comp : Switch  Criteria=u2 ~= 0  OutDataTypeStr=single
  ESO_UD_lpf : UnitDelay  SampleTime=1e-4
  ESO_UD_z1 : UnitDelay  SampleTime=1e-4
  ESO_UD_z2 : UnitDelay  SampleTime=1e-4
  G_FFB : Gain  Gain=MotorCfg.ff_b  OutDataTypeStr=single
  G_FFFc : Gain  Gain=MotorCfg.ff_fc  OutDataTypeStr=single
  G_FFJ : Gain  Gain=MotorCfg.ff_j2pikt  OutDataTypeStr=single
  PID_speed : slpidlib/PID Controller  Controller=PI  Form=Parallel  TimeDomain=Discrete-time  UseExternalTs=off  SampleTime=1e-3  IntegratorMethod=Forward Euler  FilterMethod=Forward Euler  ControllerParametersSource=internal  P=Speed_Kp  I=Speed_Ki  UseKiTs=on  D=0  UseExternalDerivativeSource=off  N=100  UseFilter=on  TunerSelectOption=Transfer Function Based (PID Tuner App)  InitialConditionSource=internal  InitialConditionForIntegrator=0  InitialConditionForFilter=0  DifferentiatorICPrevScaledInput=0  ExternalReset=none  TrackingMode=off  Kt=1  LimitOutput=on  SatLimitsSource=internal  UpperSaturationLimit=Speed_MaxOut  LowerSaturationLimit=Speed_MinOut  LinearizeAsGain=on  AntiWindupMode=back-calculation  Kb=1  LimitIntegrator=on  UpperIntegratorSaturationLimit=inf  LowerIntegratorSaturationLimit=-inf  POutMin=[]  POutMax=[]  IOutMin=[]  IOutMax=[]  DOutMin=[]  DOutMax=[]  NOutMin=[]  NOutMax=[]  SumOutMin=[]  SumOutMax=[]  SaturationOutMin=[]  SaturationOutMax=[]  PParamMin=[]  PParamMax=[]  IParamMin=[]  IParamMax=[]  DParamMin=[]  DParamMax=[]  NParamMin=[]  NParamMax=[]  KbParamMin=[]  KbParamMax=[]  KtParamMin=[]  KtParamMax=[]  KbOutMin=[]  KbOutMax=[]  KtOutMin=[]  KtOutMax=[]  IntegratorOutMin=[]  IntegratorOutMax=[]  FilterOutMin=[]  FilterOutMax=[]  SumI1OutMin=[]  SumI1OutMax=[]  SumI2OutMin=[]  SumI2OutMax=[]  SumI3OutMin=[]  SumI3OutMax=[]  SumI4OutMin=[]  SumI4OutMax=[]  SumDOutMin=[]  SumDOutMax=[]  DifferentiatorOutMin=[]  DifferentiatorOutMax=[]  FilterDiffOutCoefMin=[]  FilterDiffOutCoefMax=[]  ReciprocalOutMin=[]  ReciprocalOutMax=[]  SumDenOutMin=[]  SumDenOutMax=[]  SumNumOutMin=[]  SumNumOutMax=[]  DivideOutMin=[]  DivideOutMax=[]  UdiffTsProdOutMin=[]  UdiffTsProdOutMax=[]  NTsProdOutMin=[]  NTsProdOutMax=[]  UintegralTsProdOutMin=[]  UintegralTsProdOutMax=[]  UngainTsProdOutMin=[]  UngainTsProdOutMax=[]  ClampingZeroOutDataTypeStr=Inherit: Inherit via back propagation  ClampingZeroOutMin=[]  ClampingZeroOutMax=[]  FilterDenConstantOutDataTypeStr=Inherit: Inherit via back propagation  FilterDenConstantOutMin=[]  FilterDenConstantOutMax=[]  PCopyOutDataTypeStr=Inherit: Inherit via back propagation  PCopyOutMin=[]  PCopyOutMax=[]  NCopyOutDataTypeStr=Inherit: Inherit via back propagation  NCopyOutMin=[]  NCopyOutMax=[]  IntegratorContinuousStateAttributes=''  IntegratorStateMustResolveToSignalObject=off  IntegratorRTWStateStorageClass=Auto  FilterContinuousStateAttributes=''  FilterStateMustResolveToSignalObject=off  FilterRTWStateStorageClass=Auto  ParallelPVariant=InternalParameters  IdealPVariant=Disabled  IVariant=InternalParameters  DVariant=Disabled  IntegratorVariant=Discrete  SatVariant=Enabled  AWVariant=BackCalculation  PCopyVariant=Disabled  TRVariant=Disabled  FdbkBlocksVariant=Forward  IdealPFdbkVariant=Disabled  SatFdbkVariant=Disabled  DerivativeFilterVariant=Disabled  NVariant=Disabled  NCopyVariant=Disabled_SignalSpec  FilterICVariant=Disabled  IntegratorICVariant=InternalICs  ExternalResetVariant=Disabled  TRSumVariant=Passthrough  SumFdbkVariant=Disabled  SumVariant=Sum_PI  TsampFilterVariant=InternalTs  TsampNgainVariant=Passthrough  TsampIntegralVariant=Disabled_SignalSpec  ExternalSaturationOutDataTypeStr=Inherit: Same as second input  DerivativeSourceVariant=Disabled  PreIntVariant=InternalPreInt
  Rel_pos : RelationalOperator  Operator===  OutDataTypeStr=boolean  RndMeth=Simplest  InputSameDT=off
  Sign_FF : Signum
  Sum_FFraw : Sum  Inputs=+++  OutDataTypeStr=single
  Sum_errs : Sum  Inputs=+-
  Sum_final : Sum  Inputs=+++  OutDataTypeStr=single
  Sw_speedref : Switch  Criteria=u2 ~= 0  SaturateOnIntegerOverflow=off  InputSameDT=off
  iq_ref_speed : Outport
  wires:
  Sum_final/1 -> iq_ref_speed/1
  ESO_UD_lpf/1 -> ESO_G_lpfA/1
  ESO_G_b0/1 -> ESO_Sum_dz1/2
  ESO_Sum_e/1 -> ESO_G_b1/1, ESO_G_b2/1
  iq_meas/1 -> ESO_G_lpfB/1
  ESO_G_lpfA/1 -> ESO_Sum_lpf/1
  ESO_UD_z1/1 -> ESO_Sum_e/1, ESO_Sum_z1/2
  speed_fbk/1 -> ESO_Sum_e/2, Sum_errs/2, G_FFB/1, Sign_FF/1
  ESO_G_lpfB/1 -> ESO_Sum_lpf/2
  ESO_Sum_lpf/1 -> ESO_UD_lpf/1, ESO_G_b0/1
  Sign_FF/1 -> G_FFFc/1
  ESO_Sum_dz1/1 -> ESO_G_Ts1/1
  ref_speed/1 -> Sw_speedref/3
  ESO_G_b1/1 -> ESO_Sum_dz1/3
  ref_accel/1 -> G_FFJ/1
  G_FFB/1 -> Sum_FFraw/2
  Sw_speedref/1 -> Sum_errs/1
  speed_ref_pos/1 -> Sw_speedref/1
  Const_2/1 -> Rel_pos/2
  ctrl_mode/1 -> Rel_pos/1, ESO_Rel_mode/1
  ESO_Sum_z2/1 -> ESO_UD_z2/1
  ESO_Rel_mode/1 -> ESO_And_comp/1
  ESO_C_one/1 -> ESO_Rel_mode/2
  ESO_C_b1/1 -> ESO_Rel_b1/1
  ESO_C_b0/1 -> ESO_Rel_b0/1
  ESO_Rel_b0/1 -> ESO_And_state/1, ESO_And_comp/2
  ESO_C_zero2/1 -> ESO_Rel_b1/2
  ESO_C_zero/1 -> ESO_Rel_b0/2
  ESO_G_Ts1/1 -> ESO_P_z1/1
  ESO_Sum_dz2/1 -> ESO_G_Ts2/1
  ESO_G_b2/1 -> ESO_Sum_dz2/1
  Sum_FFraw/1 -> Sum_final/2
  G_FFFc/1 -> Sum_FFraw/3
  G_FFJ/1 -> Sum_FFraw/1
  ESO_UD_z2/1 -> ESO_Sum_dz1/1, ESO_Sum_z2/2, ESO_G_inv/1
  Rel_pos/1 -> Sw_speedref/2
  ESO_G_inv/1 -> ESO_Sum_neg/1
  ESO_Rel_b1/1 -> ESO_And_state/2, ESO_And_comp/3
  ESO_Sum_neg/1 -> ESO_Sat/1
  ESO_And_state/1 -> ESO_P_z1/2, ESO_P_z2/2
  ESO_And_comp/1 -> ESO_Sw_comp/2
  ESO_P_z1/1 -> ESO_Sum_z1/1
  ESO_G_Ts2/1 -> ESO_P_z2/1
  PID_speed/1 -> Sum_final/1
  Sum_errs/1 -> PID_speed/1
  ESO_C_zero3/1 -> ESO_Sw_comp/3
  ESO_Sat/1 -> ESO_Sw_comp/1
  ESO_Sum_z1/1 -> ESO_UD_z1/1
  ESO_P_z2/1 -> ESO_Sum_z2/1
  ESO_Sw_comp/1 -> Sum_final/3
